simulink model "ControllerCore"  (R2026b)
settings: Solver=VariableStepAuto
settings Model: Creator=fayne  LastModifiedBy=fayne

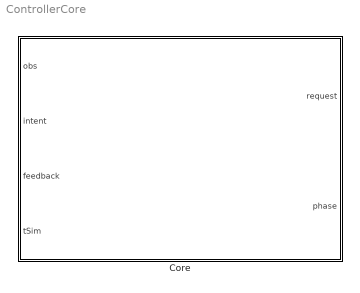
== system ControllerCore ==
  Core : Subsystem

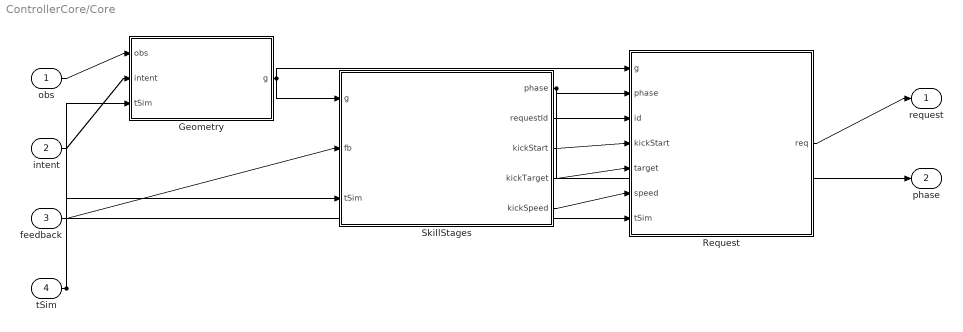
== system ControllerCore/Core ==
  obs : Inport
  intent : Inport  Port=2
  feedback : Inport  Port=3
  tSim : Inport  Port=4
  Geometry : MATLAB Function  TreatAsAtomicUnit=on
  Request : MATLAB Function  TreatAsAtomicUnit=on
  SkillStages : Stateflow chart  TreatAsAtomicUnit=on
  request : Outport
  phase : Outport  Port=2
  wires:
  obs/1 -> Geometry/1(obs)
  intent/1 -> Geometry/2(intent)
  tSim/1 -> Geometry/3(tSim), SkillStages/3(tSim), Request/7(tSim)
  Geometry/1(g) -> SkillStages/1(g), Request/1(g)
  feedback/1 -> SkillStages/2(fb)
  SkillStages/1(phase) -> Request/2(phase), phase/1
  SkillStages/2(requestId) -> Request/3(id)
  SkillStages/3(kickStart) -> Request/4(kickStart)
  SkillStages/4(kickTarget) -> Request/5(target)
  SkillStages/5(kickSpeed) -> Request/6(speed)
  Request/1(req) -> request/1

== matlab function ControllerCore/Core/Request ==
  data: g input Bus: GeometryBus; req output Bus: RequestBus; phase input Enum: TdpPhase; id input uint32; kickStart input; target input; speed input; tSim input; P parameter
function req=f(g,phase,id,kickStart,target,speed,tSim,P)
req=EmitRequest(g,phase,id,kickStart,target,speed,tSim,P);
end

== matlab function ControllerCore/Core/Geometry ==
  data: obs input Bus: ObservationBus; g output Bus: GeometryBus; intent input Bus: IntentBus; tSim input; P parameter
function g=f(obs,intent,tSim,P)
g=CoreGeometry(obs,intent,tSim,P);
end

== stateflow chart ControllerCore/Core/SkillStages ==
  settings: updateMethod=DISCRETE  sampleTime=P.dt
  state Idle
    en,du:
    phase=TdpPhase.Idle;
    requestId=requestId+uint32(1);
  state Active
    en,du:
    if P.mode==TdpMode.Compat || phase~=TdpPhase.Kick
    requestId=requestId+uint32(1);
    end
    state Search
      en: phase=TdpPhase.Search;
    state Approach
      en: phase=TdpPhase.Approach;
    state Align
      en: phase=TdpPhase.Align;
    state Kick
      en:
      phase=TdpPhase.Kick;
      requestId=requestId+uint32(1);
      kickStart=tSim;
      kickTarget=g.target;
      kickSpeed=g.speed;
    state Recover
      en:
      phase=TdpPhase.Recover;
      recoverStart=tSim;
    (default) -> Search
    Align -> Kick [order 3] : [g.ready]
    Align -> Search [order 1] : [~g.ballVisible]
    Approach -> Search [order 1] : [~g.ballVisible && g.intent~=TdpAction.Goto]
    Recover -> Search : [tSim-recoverStart>=P.recoverTime]
    Search -> Approach : [g.ballVisible || g.intent==TdpAction.Goto]
    Align -> Approach [order 2] : [g.distance>P.alignExit || g.intent==TdpAction.Goto]
    Approach -> Align [order 2] : [g.distance<P.alignEnter && g.intent~=TdpAction.Goto]
    Kick -> Recover [order 1] : [fb.requestId==requestId && (fb.status==TdpStatus.Done || fb.status==TdpStatus.Failed || fb.status==TdpStatus.Rejected)]
    Kick -> Recover [order 2] : [tSim-kickStart>=P.kickTimeout]
    Kick -> Recover [order 3] : [~g.ballVisible]
  (default) -> Idle : {requestId=uint32(0);kickStart=0;kickTarget=[0 0];kickSpeed=0;recoverStart=0;}
  Active -> Idle : [~g.safe || (~g.running && P.mode==TdpMode.Delayed)]
  Idle -> Active : [g.safe && (g.running || P.mode==TdpMode.Compat)]
  data: g input Bus: GeometryBus size=1; fb input Bus: FeedbackBus size=1; tSim input double size=1; P parameter size=1; phase output Enum: TdpPhase size=1; requestId output uint32 size=1; kickStart output double size=1; kickTarget output double size=[1 2]; kickSpeed output double size=1; recoverStart local double size=1
